simulink model "gauss_markov"  (Simulink 9.1)
settings: Solver=ode45  StartTime=0.0  StopTime=10.0  RelTol=1e-3  EnableMultiTasking=on
libraries: simulink x1
settings Model: Creator=mcar  LastModifiedBy=1104070
settings DataIOCC: LimitDataPoints=on  SignalLoggingSaveFormat=ModelDataLogs
settings OptimizationCC: BlockReduction=off  BooleanDataType=off  LifeSpan=auto
settings DebuggingCC: SaveWithParameterizedLinksMsg=none  SignalResolutionControl=TryResolveAllWithWarning  MultiTaskDSMMsg=warning  MultiTaskCondExecSysMsg=none  SFUnexpectedBacktrackingDiag=error  SFNoUnconditionalDefaultTransitionDiag=error  SFExecutionAtInitializationDiag=warning
settings HardwareCC: ProdBitPerPointer=64  ProdBitPerSizeT=64  ProdBitPerPtrDiffT=64  ProdLargestAtomicFloat=Float  ProdIntDivRoundTo=Zero  ProdEndianess=LittleEndian  ProdWordSize=64  ProdHWDeviceType=Intel->x86-64 (Windows64)  TargetUnknown=on
settings CodeAppCC: StateflowObjectComments=off
settings ConfigComp: CovMetricSettings=dwe

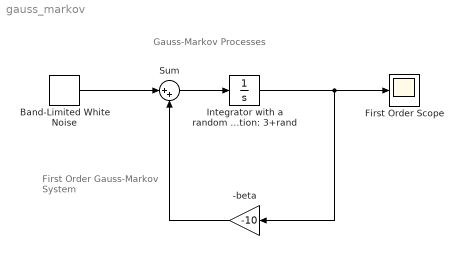
== system gauss_markov ==
  note: Gauss-Markov Processes
  note: First Order
      | Gauss-Markov System
  -beta : Gain  Gain=-10  SaturateOnIntegerOverflow=on  OutDataTypeStr=Inherit: Same as input  ParamDataTypeStr=Inherit: Same as input
  Band-Limited White Noise : simulink/Sources/Band-Limited White Noise  Cov=[10]  Ts=0.01  seed=[23341]
  First Order Scope : Scope
  Integrator with a random initial condition: 3+rand : Integrator
  Sum : Sum  Inputs=|++  SaturateOnIntegerOverflow=on  InputSameDT=on  OutDataTypeStr=Inherit: Same as first input
  wires:
  Integrator with a random initial condition: 3+rand/1 -> -beta/1, First Order Scope/1
  -beta/1 -> Sum/2
  Sum/1 -> Integrator with a random initial condition: 3+rand/1
  Band-Limited White Noise/1 -> Sum/1
